simulink model "decodeur_hamming"  (R2023b)
settings: Solver=FixedStepDiscrete  StartTime=0.0  StopTime=127  FixedStep=1  RelTol=1e-3
settings Model: Creator=e2507477  LastModifiedBy=e2507477

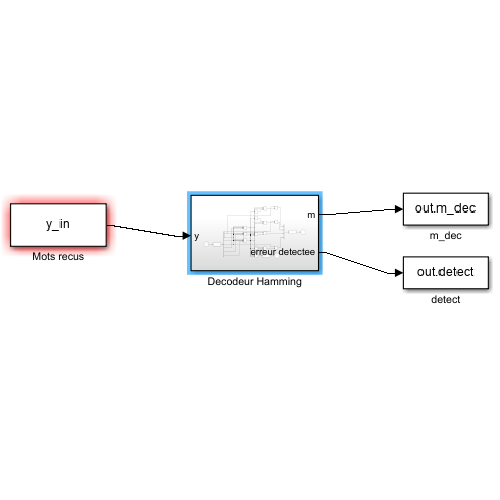
[thumbnail: Simulink's stored preview of the top-level diagram]
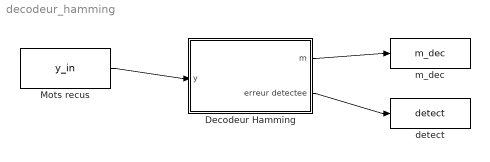
== system decodeur_hamming ==
  Decodeur Hamming : Subsystem
  Mots recus : FromWorkspace  VariableName=y_in  SampleTime=1  Interpolate=off  OutputAfterFinalValue=Holding final value
  detect : ToWorkspace  VariableName=detect  SampleTime=-1
  m_dec : ToWorkspace  VariableName=m_dec  SampleTime=-1
  wires:
  Mots recus/1 -> Decodeur Hamming/1(y)
  Decodeur Hamming/1(m) -> m_dec/1
  Decodeur Hamming/2(erreur detectee) -> detect/1

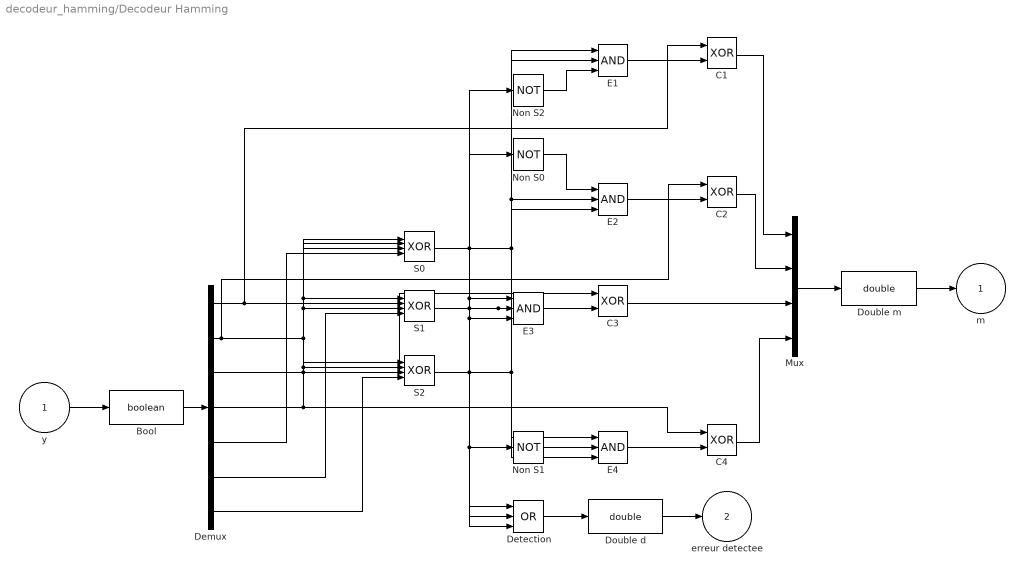
== system decodeur_hamming/Decodeur Hamming ==
  y : Inport
  Bool : DataTypeConversion  OutDataTypeStr=boolean  SaturateOnIntegerOverflow=off  RndMeth=Floor
  C{1..4} (4 alike) : Logic  Operator=XOR  AllPortsSameDT=off  OutDataTypeStr=boolean
  Demux : Demux  Outputs=7
  Detection : Logic  Operator=OR  Inputs=3  AllPortsSameDT=off  OutDataTypeStr=boolean
  Double d : DataTypeConversion  OutDataTypeStr=double  SaturateOnIntegerOverflow=off  RndMeth=Floor
  Double m : DataTypeConversion  OutDataTypeStr=double  SaturateOnIntegerOverflow=off  RndMeth=Floor
  E{1..4} (4 alike) : Logic  Inputs=3  AllPortsSameDT=off  OutDataTypeStr=boolean
  Mux : Mux
  Non S0 : Logic  Operator=NOT  AllPortsSameDT=off  OutDataTypeStr=boolean
  Non S1 : Logic  Operator=NOT  AllPortsSameDT=off  OutDataTypeStr=boolean
  Non S2 : Logic  Operator=NOT  AllPortsSameDT=off  OutDataTypeStr=boolean
  S0 : Logic  Operator=XOR  Inputs=4  AllPortsSameDT=off  OutDataTypeStr=boolean
  S1 : Logic  Operator=XOR  Inputs=4  AllPortsSameDT=off  OutDataTypeStr=boolean
  S2 : Logic  Operator=XOR  Inputs=4  AllPortsSameDT=off  OutDataTypeStr=boolean
  m : Outport
  erreur detectee : Outport  Port=2
  wires:
  Demux/4 -> S0/3, S2/3, C4/1
  Non S1/1 -> E4/2
  Non S0/1 -> E2/1
  Demux/2 -> S2/1, S1/2, C2/1
  Bool/1 -> Demux/1
  y/1 -> Bool/1
  Demux/6 -> S1/4
  Demux/3 -> S0/2, S1/3, S2/2, C3/1
  Demux/1 -> S0/1, S1/1, C1/1
  Detection/1 -> Double d/1
  Demux/5 -> S0/4
  S1/1 -> Non S1/1, Detection/2, E1/2, E2/2, E3/2
  S0/1 -> Detection/1, E3/1, E1/1, E4/1, Non S0/1
  Demux/7 -> S2/4
  S2/1 -> E2/3, E4/3, E3/3, Non S2/1, Detection/3
  Non S2/1 -> E1/3
  E3/1 -> C3/2
  E1/1 -> C1/2
  E2/1 -> C2/2
  C3/1 -> Mux/3
  E4/1 -> C4/2
  Double d/1 -> erreur detectee/1
  C1/1 -> Mux/1
  C2/1 -> Mux/2
  C4/1 -> Mux/4
  Mux/1 -> Double m/1
  Double m/1 -> m/1
